simulink model "Roll_Pitch_Controller_AW"  (R2026b)
settings: Solver=FixedStepDiscrete  FixedStep=0.01  EnableMultiTasking=on
libraries: slpidlib x2
settings OptimizationCC: DefaultParameterBehavior=Inlined  DifferentSizesBufferReuse=on  EfficientTunableParamExpr=on  EnhancedBackFolding=on  MaxStackSize=512  OptimizationCustomize=off  OptimizeBlockOrder=speed  PassReuseOutputArgsAs=Individual arguments  RemoveInternalMemoryZeroInit=on  RemoveRootLevelIOMemoryZeroInit=on
settings DebuggingCC: ParameterTunabilityLossMsg=error
settings SFSimCC: MATLABDynamicMemAlloc=off
settings RTWCC: BuildConfiguration=Faster Runs  DataTypeReplacement=CDataTypesFixedWidth  Description=Embedded Coder  SystemTargetFile=ert.tlc  TemplateMakefile=ert_default_tmf  Toolchain=MinGW64 | gmake (64-bit Windows)
settings CodeAppCC: ForceParamTrailComments=on  IgnoreCustomStorageClasses=off  InsertBlockDesc=on  OperatorAnnotations=on  SFDataObjDesc=on  SimulinkDataObjDesc=on
settings ERTTargetCC: CombineSignalStateStructs=on  ExtModeIntrfLevel=Level2 - Open  ExtModeMexFile=ext_xcp  ExtModeStaticAlloc=on  MaxIdInt16=INT16_MAX  MaxIdInt32=INT32_MAX  MaxIdInt64=INT64_MAX  MaxIdInt8=INT8_MAX  MaxIdUint16=UINT16_MAX  MaxIdUint32=UINT32_MAX  MaxIdUint64=UINT64_MAX  MaxIdUint8=UINT8_MAX  MinIdInt16=INT16_MIN  MinIdInt32=INT32_MIN  MinIdInt64=INT64_MIN  MinIdInt8=INT8_MIN

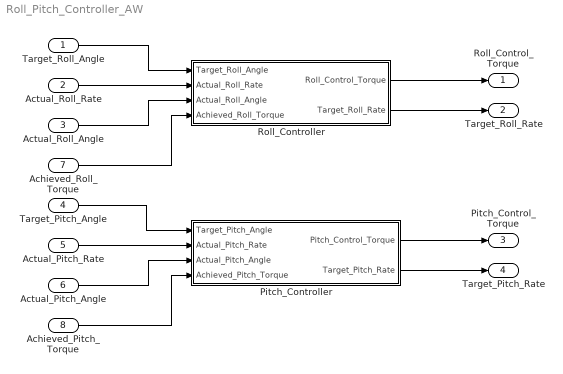
== system Roll_Pitch_Controller_AW ==
  Target_Roll_Angle : Inport  OutDataTypeStr=single
  Actual_Roll_Rate : Inport  Port=2  OutDataTypeStr=single
  Actual_Roll_Angle : Inport  Port=3  OutDataTypeStr=single
  Target_Pitch_Angle : Inport  Port=4
  Actual_Pitch_Rate : Inport  Port=5
  Actual_Pitch_Angle : Inport  Port=6  OutDataTypeStr=single
  Achieved_Roll_Torque : Inport  Port=7  OutDataTypeStr=single
  Achieved_Pitch_Torque : Inport  Port=8  OutDataTypeStr=single
  Pitch_Controller : Subsystem
  Roll_Controller : Subsystem
  Roll_Control_Torque : Outport  OutDataTypeStr=single
  Target_Roll_Rate : Outport  Port=2  OutDataTypeStr=single
  Pitch_Control_Torque : Outport  Port=3  OutDataTypeStr=single
  Target_Pitch_Rate : Outport  Port=4  OutDataTypeStr=single
  wires:
  Target_Roll_Angle/1 -> Roll_Controller/1(Target_Roll_Angle)
  Actual_Roll_Rate/1 -> Roll_Controller/2(Actual_Roll_Rate)
  Actual_Roll_Angle/1 -> Roll_Controller/3(Actual_Roll_Angle)
  Actual_Pitch_Rate/1 -> Pitch_Controller/2(Actual_Pitch_Rate)
  Actual_Pitch_Angle/1 -> Pitch_Controller/3(Actual_Pitch_Angle)
  Target_Pitch_Angle/1 -> Pitch_Controller/1(Target_Pitch_Angle)
  Roll_Controller/1(Roll_Control_Torque) -> Roll_Control_Torque/1
  Roll_Controller/2(Target_Roll_Rate) -> Target_Roll_Rate/1
  Pitch_Controller/2(Target_Pitch_Rate) -> Target_Pitch_Rate/1
  Pitch_Controller/1(Pitch_Control_Torque) -> Pitch_Control_Torque/1
  Achieved_Roll_Torque/1 -> Roll_Controller/4(Achieved_Roll_Torque)
  Achieved_Pitch_Torque/1 -> Pitch_Controller/4(Achieved_Pitch_Torque)

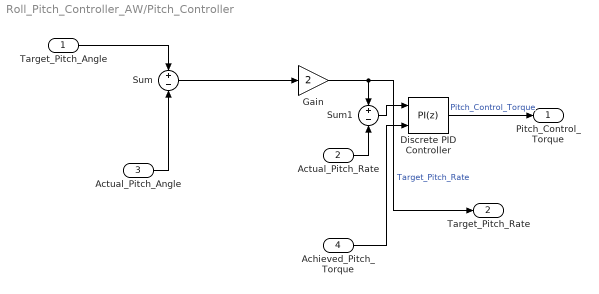
== system Roll_Pitch_Controller_AW/Pitch_Controller ==
  Target_Pitch_Angle : Inport
  Actual_Pitch_Rate : Inport  Port=2
  Actual_Pitch_Angle : Inport  Port=3
  Achieved_Pitch_Torque : Inport  Port=4  OutDataTypeStr=single
  Discrete PID Controller : slpidlib/PID Controller  Controller=PI  Form=Parallel  TimeDomain=Discrete-time  UseExternalTs=off  SampleTime=0.01  IntegratorMethod=Forward Euler  FilterMethod=Forward Euler  ControllerParametersSource=internal  P=0.05  I=0.2  UseKiTs=off  D=0  UseExternalDerivativeSource=off  N=100  UseFilter=on  TunerSelectOption=Transfer Function Based (PID Tuner App)  InitialConditionSource=internal  InitialConditionForIntegrator=0  InitialConditionForFilter=0  DifferentiatorICPrevScaledInput=0  ExternalReset=none  TrackingMode=on  Kt=2  LimitOutput=off  SatLimitsSource=internal  UpperSaturationLimit=inf  LowerSaturationLimit=-inf  LinearizeAsGain=off  AntiWindupMode=none  Kb=1  LimitIntegrator=off  UpperIntegratorSaturationLimit=inf  LowerIntegratorSaturationLimit=-inf  POutMin=[]  POutMax=[]  IOutMin=[]  IOutMax=[]  DOutMin=[]  DOutMax=[]  NOutMin=[]  NOutMax=[]  SumOutMin=[]  SumOutMax=[]  SaturationOutMin=[]  SaturationOutMax=[]  PParamMin=[]  PParamMax=[]  IParamMin=[]  IParamMax=[]  DParamMin=[]  DParamMax=[]  NParamMin=[]  NParamMax=[]  KbParamMin=[]  KbParamMax=[]  KtParamMin=[]  KtParamMax=[]  KbOutMin=[]  KbOutMax=[]  KtOutMin=[]  KtOutMax=[]  IntegratorOutMin=[]  IntegratorOutMax=[]  FilterOutMin=[]  FilterOutMax=[]  SumI1OutMin=[]  SumI1OutMax=[]  SumI2OutMin=[]  SumI2OutMax=[]  SumI3OutMin=[]  SumI3OutMax=[]  SumI4OutMin=[]  SumI4OutMax=[]  SumDOutMin=[]  SumDOutMax=[]  DifferentiatorOutMin=[]  DifferentiatorOutMax=[]  FilterDiffOutCoefMin=[]  FilterDiffOutCoefMax=[]  ReciprocalOutMin=[]  ReciprocalOutMax=[]  SumDenOutMin=[]  SumDenOutMax=[]  SumNumOutMin=[]  SumNumOutMax=[]  DivideOutMin=[]  DivideOutMax=[]  UdiffTsProdOutMin=[]  UdiffTsProdOutMax=[]  NTsProdOutMin=[]  NTsProdOutMax=[]  UintegralTsProdOutMin=[]  UintegralTsProdOutMax=[]  UngainTsProdOutMin=[]  UngainTsProdOutMax=[]  ClampingZeroOutDataTypeStr=Inherit: Inherit via back propagation  ClampingZeroOutMin=[]  ClampingZeroOutMax=[]  FilterDenConstantOutDataTypeStr=Inherit: Inherit via back propagation  FilterDenConstantOutMin=[]  FilterDenConstantOutMax=[]  PCopyOutDataTypeStr=Inherit: Inherit via back propagation  PCopyOutMin=[]  PCopyOutMax=[]  NCopyOutDataTypeStr=Inherit: Inherit via back propagation  NCopyOutMin=[]  NCopyOutMax=[]  IntegratorContinuousStateAttributes=''  IntegratorStateMustResolveToSignalObject=off  IntegratorRTWStateStorageClass=Auto  FilterContinuousStateAttributes=''  FilterStateMustResolveToSignalObject=off  FilterRTWStateStorageClass=Auto  ParallelPVariant=InternalParameters  IdealPVariant=Disabled  IVariant=InternalParameters  DVariant=Disabled  IntegratorVariant=Discrete  SatVariant=Disabled  AWVariant=Passthrough  PCopyVariant=Disabled  TRVariant=Enabled  FdbkBlocksVariant=Forward  IdealPFdbkVariant=Disabled  SatFdbkVariant=Disabled  DerivativeFilterVariant=Disabled  NVariant=Disabled  NCopyVariant=Disabled_SignalSpec  FilterICVariant=Disabled  IntegratorICVariant=InternalICs  ExternalResetVariant=Disabled  TRSumVariant=TrackingMode  SumFdbkVariant=Disabled  SumVariant=Sum_PI  TsampFilterVariant=InternalTs  TsampNgainVariant=Passthrough  TsampIntegralVariant=Disabled_SignalSpec  ExternalSaturationOutDataTypeStr=Inherit: Same as second input  DerivativeSourceVariant=Disabled  PreIntVariant=InternalPreInt
      settings: LibrarySourceBlock=simulink/Discrete/Discrete PID Controller
  Gain : Gain  Gain=2
  Sum : Sum  Inputs=+-
  Sum1 : Sum  Inputs=+-
  Pitch_Control_Torque : Outport
  Target_Pitch_Rate : Outport  Port=2
  wires:
  Actual_Pitch_Rate/1 -> Sum1/2
  Gain/1 -> Target_Pitch_Rate/1, Sum1/1  "Target_Pitch_Rate"
  Target_Pitch_Angle/1 -> Sum/1
  Sum/1 -> Gain/1
  Actual_Pitch_Angle/1 -> Sum/2
  Sum1/1 -> Discrete PID Controller/1
  Discrete PID Controller/1 -> Pitch_Control_Torque/1  "Pitch_Control_Torque"
  Achieved_Pitch_Torque/1 -> Discrete PID Controller/2

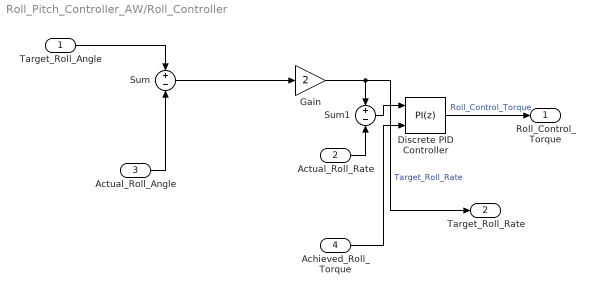
== system Roll_Pitch_Controller_AW/Roll_Controller ==
  Target_Roll_Angle : Inport  OutDataTypeStr=single
  Actual_Roll_Rate : Inport  Port=2  OutDataTypeStr=single
  Actual_Roll_Angle : Inport  Port=3  OutDataTypeStr=single
  Achieved_Roll_Torque : Inport  Port=4  OutDataTypeStr=single
  Discrete PID Controller : slpidlib/PID Controller  Controller=PI  Form=Parallel  TimeDomain=Discrete-time  UseExternalTs=off  SampleTime=0.01  IntegratorMethod=Forward Euler  FilterMethod=Forward Euler  ControllerParametersSource=internal  P=0.05  I=0.2  UseKiTs=off  D=0  UseExternalDerivativeSource=off  N=100  UseFilter=on  TunerSelectOption=Transfer Function Based (PID Tuner App)  InitialConditionSource=internal  InitialConditionForIntegrator=0  InitialConditionForFilter=0  DifferentiatorICPrevScaledInput=0  ExternalReset=none  TrackingMode=on  Kt=2  LimitOutput=off  SatLimitsSource=internal  UpperSaturationLimit=inf  LowerSaturationLimit=-inf  LinearizeAsGain=off  AntiWindupMode=none  Kb=1  LimitIntegrator=off  UpperIntegratorSaturationLimit=inf  LowerIntegratorSaturationLimit=-inf  POutMin=[]  POutMax=[]  IOutMin=[]  IOutMax=[]  DOutMin=[]  DOutMax=[]  NOutMin=[]  NOutMax=[]  SumOutMin=[]  SumOutMax=[]  SaturationOutMin=[]  SaturationOutMax=[]  PParamMin=[]  PParamMax=[]  IParamMin=[]  IParamMax=[]  DParamMin=[]  DParamMax=[]  NParamMin=[]  NParamMax=[]  KbParamMin=[]  KbParamMax=[]  KtParamMin=[]  KtParamMax=[]  KbOutMin=[]  KbOutMax=[]  KtOutMin=[]  KtOutMax=[]  IntegratorOutMin=[]  IntegratorOutMax=[]  FilterOutMin=[]  FilterOutMax=[]  SumI1OutMin=[]  SumI1OutMax=[]  SumI2OutMin=[]  SumI2OutMax=[]  SumI3OutMin=[]  SumI3OutMax=[]  SumI4OutMin=[]  SumI4OutMax=[]  SumDOutMin=[]  SumDOutMax=[]  DifferentiatorOutMin=[]  DifferentiatorOutMax=[]  FilterDiffOutCoefMin=[]  FilterDiffOutCoefMax=[]  ReciprocalOutMin=[]  ReciprocalOutMax=[]  SumDenOutMin=[]  SumDenOutMax=[]  SumNumOutMin=[]  SumNumOutMax=[]  DivideOutMin=[]  DivideOutMax=[]  UdiffTsProdOutMin=[]  UdiffTsProdOutMax=[]  NTsProdOutMin=[]  NTsProdOutMax=[]  UintegralTsProdOutMin=[]  UintegralTsProdOutMax=[]  UngainTsProdOutMin=[]  UngainTsProdOutMax=[]  ClampingZeroOutDataTypeStr=Inherit: Inherit via back propagation  ClampingZeroOutMin=[]  ClampingZeroOutMax=[]  FilterDenConstantOutDataTypeStr=Inherit: Inherit via back propagation  FilterDenConstantOutMin=[]  FilterDenConstantOutMax=[]  PCopyOutDataTypeStr=Inherit: Inherit via back propagation  PCopyOutMin=[]  PCopyOutMax=[]  NCopyOutDataTypeStr=Inherit: Inherit via back propagation  NCopyOutMin=[]  NCopyOutMax=[]  IntegratorContinuousStateAttributes=''  IntegratorStateMustResolveToSignalObject=off  IntegratorRTWStateStorageClass=Auto  FilterContinuousStateAttributes=''  FilterStateMustResolveToSignalObject=off  FilterRTWStateStorageClass=Auto  ParallelPVariant=InternalParameters  IdealPVariant=Disabled  IVariant=InternalParameters  DVariant=Disabled  IntegratorVariant=Discrete  SatVariant=Disabled  AWVariant=Passthrough  PCopyVariant=Disabled  TRVariant=Enabled  FdbkBlocksVariant=Forward  IdealPFdbkVariant=Disabled  SatFdbkVariant=Disabled  DerivativeFilterVariant=Disabled  NVariant=Disabled  NCopyVariant=Disabled_SignalSpec  FilterICVariant=Disabled  IntegratorICVariant=InternalICs  ExternalResetVariant=Disabled  TRSumVariant=TrackingMode  SumFdbkVariant=Disabled  SumVariant=Sum_PI  TsampFilterVariant=InternalTs  TsampNgainVariant=Passthrough  TsampIntegralVariant=Disabled_SignalSpec  ExternalSaturationOutDataTypeStr=Inherit: Same as second input  DerivativeSourceVariant=Disabled  PreIntVariant=InternalPreInt
      settings: LibrarySourceBlock=simulink/Discrete/Discrete PID Controller
  Gain : Gain  Gain=2
  Sum : Sum  Inputs=+-
  Sum1 : Sum  Inputs=+-
  Roll_Control_Torque : Outport
  Target_Roll_Rate : Outport  Port=2
  wires:
  Discrete PID Controller/1 -> Roll_Control_Torque/1  "Roll_Control_Torque"
  Sum1/1 -> Discrete PID Controller/1
  Actual_Roll_Rate/1 -> Sum1/2
  Sum/1 -> Gain/1
  Gain/1 -> Target_Roll_Rate/1, Sum1/1  "Target_Roll_Rate"
  Actual_Roll_Angle/1 -> Sum/2
  Target_Roll_Angle/1 -> Sum/1
  Achieved_Roll_Torque/1 -> Discrete PID Controller/2
